simulink model "pwm_test"  (R2024b)
settings: Solver=FixedStepDiscrete  StartTime=0.0  StopTime=inf  FixedStep=0.001  RelTol=1e-3
undefined symbols (not defined in the file): ESP32, Levenberg, Marquardt, waypoints, WROOM, X, Y, Z
libraries: sm_lib x46, nesl_utility x13, arduinolib x6, simulink x5, robotcorelib x1, robotmaniplib x1, simulink_extras x1
(part 2 of 2)

== system pwm_test/Plant/Arm/link_6 ==
  AxisTransform revolute link_6 : sm_lib/Frames and Transforms/Rigid Transform  RotationMethod=StandardAxis  FollAlignAxisA=+X  BaseAlignAxisA=+Y  FollAlignAxisB=+Y  BaseAlignAxisB=+Z  RotationStandardAxis=+Y  RotationAngle=90  RotationAngleUnits=deg  RotationArbitraryAxis=[0 0 1]  RotationSequenceAxes=FollowerAxes  RotationSequence=XYZ  RotationSequenceAngles=[0 0 119.162]  RotationSequenceAnglesUnits=deg  RotationMatrix=[0 0 0; 0 0 0; 0 0 0]  Quaternion=[1 0 0 0]  TranslationMethod=None  TranslationCartesianOffset=[0 0 0]  TranslationCartesianOffsetUnits=m  TranslationStandardAxis=+Z  TranslationStandardOffset=0  TranslationStandardOffsetUnits=m  TranslationROffset=0  TranslationROffsetUnits=m  TranslationThetaOffset=0  TranslationThetaOffsetUnits=deg  TranslationZOffset=0  TranslationZOffsetUnits=m
  OriginTransform revolute link_6 : sm_lib/Frames and Transforms/Rigid Transform  RotationMethod=None  FollAlignAxisA=+X  BaseAlignAxisA=+Y  FollAlignAxisB=+Y  BaseAlignAxisB=+Z  RotationStandardAxis=+Z  RotationAngle=0  RotationAngleUnits=deg  RotationArbitraryAxis=[0 0 1]  RotationSequenceAxes=FollowerAxes  RotationSequence=XYX  RotationSequenceAngles=[0 0 0]  RotationSequenceAnglesUnits=deg  RotationMatrix=[1 0 0;0 1 0;0 0 1]  Quaternion=[1 0 0 0]  TranslationMethod=Cartesian  TranslationCartesianOffset=[9.367 0.00 43.933]  TranslationCartesianOffsetUnits=mm  TranslationStandardAxis=+Z  TranslationStandardOffset=0  TranslationStandardOffsetUnits=m  TranslationROffset=0  TranslationROffsetUnits=m  TranslationThetaOffset=0  TranslationThetaOffsetUnits=deg  TranslationZOffset=0  TranslationZOffsetUnits=m
  Reference Frame : sm_lib/Frames and Transforms/Reference Frame
  link_5 : sm_lib/Body Elements/File Solid  ExtGeomFileName=./meshes/link_5.stl  UnitType=Custom  ExtGeomFileUnits=mm  StepReaderType=HEX  ExportConvexHullGeometry=off  InertiaType=CalculateFromGeometry  BasedOnType=Mass  Density=7986.89  DensityUnits=kg/m^3  Mass=680.695  MassUnits=g  CenterOfMass=[0.00, 0.00, 7.613]  CenterOfMassUnits=mm  MomentsOfInertia=[1 1 1]  MomentsOfInertiaUnits=g*mm^2  ProductsOfInertia=[0 0 0]  ProductsOfInertiaUnits=g*mm^2  GraphicType=FromGeometry  MarkerShape=Sphere  MarkerSize=10  GraphicVisPropType=SimpleVisualProperties  GraphicDiffuseColor=[0.5 0.5 0.5]  GraphicOpacity=1.0  GraphicSpecularColor=[0.5 0.5 0.5 1.0]  GraphicAmbientColor=[0.15 0.15 0.15 1.0]  GraphicEmissiveColor=[0.0 0.0 0.0 1.0]  GraphicShininess=75  DoExposeReferenceFrame=on  SerializedFrames=<Frames/>
  joint 5 : PMIOPort  Side=Left
  joint 6 : PMIOPort  Port=2  Side=Right
  connections:
  joint 6/RConn1 -- AxisTransform revolute link_6/RConn1
  AxisTransform revolute link_6/LConn1 -- OriginTransform revolute link_6/RConn1
  link_5/RConn1 -- Reference Frame/RConn1 -- joint 5/RConn1 -- OriginTransform revolute link_6/LConn1

== system pwm_test/Plant/Arm/link_7 ==
  Reference Frame : sm_lib/Frames and Transforms/Reference Frame
  link_7 : sm_lib/Body Elements/File Solid  ExtGeomFileName=./meshes/link_7.stl  UnitType=Custom  ExtGeomFileUnits=mm  StepReaderType=HEX  ExportConvexHullGeometry=off  InertiaType=CalculateFromGeometry  BasedOnType=Mass  Density=7986.89  DensityUnits=kg/m^3  Mass=680.695  MassUnits=g  CenterOfMass=[0.00, 0.00, 7.613]  CenterOfMassUnits=mm  MomentsOfInertia=[1 1 1]  MomentsOfInertiaUnits=g*mm^2  ProductsOfInertia=[0 0 0]  ProductsOfInertiaUnits=g*mm^2  GraphicType=FromGeometry  MarkerShape=Sphere  MarkerSize=10  GraphicVisPropType=SimpleVisualProperties  GraphicDiffuseColor=[0.5 0.5 0.5]  GraphicOpacity=1.0  GraphicSpecularColor=[0.5 0.5 0.5 1.0]  GraphicAmbientColor=[0.15 0.15 0.15 1.0]  GraphicEmissiveColor=[0.0 0.0 0.0 1.0]  GraphicShininess=75  DoExposeReferenceFrame=on  SerializedFrames=<Frames/>
  joint 6 : PMIOPort  Side=Left
  connections:
  joint 6/RConn1 -- Reference Frame/RConn1 -- link_7/RConn1
